simulink model "drone_controller"  (R2026b)
settings: Solver=FixedStepDiscrete  StopTime=0.1  FixedStep=Ts_Rate
model workspace (MAT data in the model file):
  Command_Max = 1
  Kp_Rate = 0.1
  Kp_Tilt = 4
  Quad_X_Mix = [-0.5  0.5  0.5; -0.5  -0.5  -0.5; 0.5  -0.5  0.5; 0.5  0.5  -0.5]
  Quaternion_Norm_Sq_Tol = 0.02
  Rate_Max_radps = 2
  Tilt_Max_rad = 0.436332312999
  Ts_Attitude = 0.01
  Ts_Rate = 0.002
libraries: simulink x6
settings Model: Creator=ASUS  LastModifiedBy=ASUS

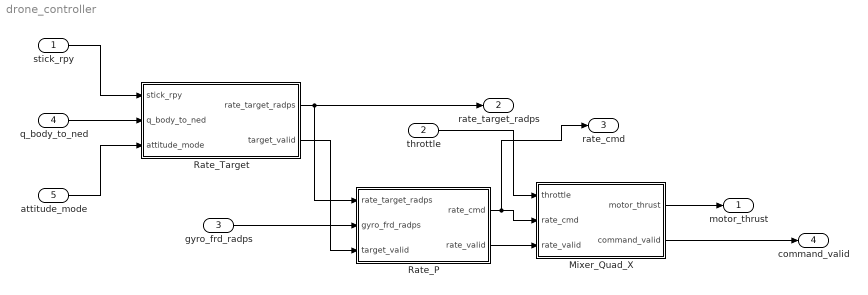
== system drone_controller ==
  stick_rpy : Inport  OutDataTypeStr=double  PortDimensions=3  SampleTime=Ts_Rate  Interpolate=off
  throttle : Inport  Port=2  OutDataTypeStr=double  PortDimensions=1  SampleTime=Ts_Rate  Interpolate=off
  gyro_frd_radps : Inport  Port=3  OutDataTypeStr=double  PortDimensions=3  SampleTime=Ts_Rate  Interpolate=off
  q_body_to_ned : Inport  Port=4  OutDataTypeStr=double  PortDimensions=4  SampleTime=Ts_Rate  Interpolate=off
  attitude_mode : Inport  Port=5  OutDataTypeStr=boolean  PortDimensions=1  SampleTime=Ts_Rate  Interpolate=off
  Mixer_Quad_X : Subsystem
  Rate_P : Subsystem
  Rate_Target : Subsystem
  motor_thrust : Outport
  rate_target_radps : Outport  Port=2
  rate_cmd : Outport  Port=3
  command_valid : Outport  Port=4
  wires:
  stick_rpy/1 -> Rate_Target/1(stick_rpy)
  q_body_to_ned/1 -> Rate_Target/2(q_body_to_ned)
  attitude_mode/1 -> Rate_Target/3(attitude_mode)
  Rate_Target/1(rate_target_radps) -> Rate_P/1(rate_target_radps), rate_target_radps/1
  gyro_frd_radps/1 -> Rate_P/2(gyro_frd_radps)
  Rate_Target/2(target_valid) -> Rate_P/3(target_valid)
  throttle/1 -> Mixer_Quad_X/1(throttle)
  Rate_P/1(rate_cmd) -> Mixer_Quad_X/2(rate_cmd), rate_cmd/1
  Rate_P/2(rate_valid) -> Mixer_Quad_X/3(rate_valid)
  Mixer_Quad_X/1(motor_thrust) -> motor_thrust/1
  Mixer_Quad_X/2(command_valid) -> command_valid/1

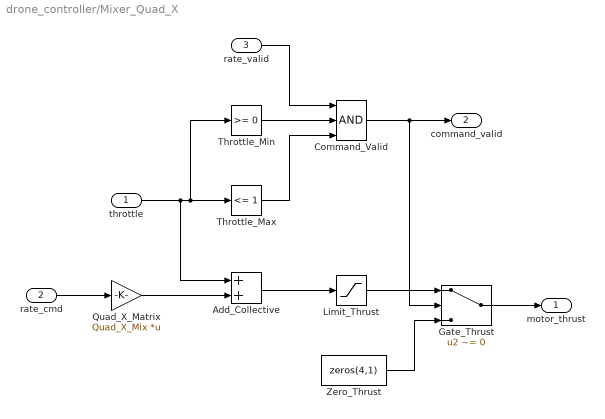
== system drone_controller/Mixer_Quad_X ==
  throttle : Inport
  rate_cmd : Inport  Port=2
  rate_valid : Inport  Port=3
  Add_Collective : Sum
  Command_Valid : Logic  Inputs=3  IconShape=distinctive  AllPortsSameDT=off  OutDataTypeStr=boolean
  Gate_Thrust : Switch  Criteria=u2 ~= 0  SaturateOnIntegerOverflow=off  InputSameDT=off
  Limit_Thrust : Saturate  UpperLimit=1  LowerLimit=0
  Quad_X_Matrix : Gain  Gain=Quad_X_Mix  Multiplication=Matrix(K*u) (u vector)
  Throttle_Max : simulink/Logic and Bit Operations/Compare To Constant  relop=<=  const=1  OutDataTypeStr=boolean
  Throttle_Min : simulink/Logic and Bit Operations/Compare To Constant  relop=>=  const=0  OutDataTypeStr=boolean
  Zero_Thrust : Constant  Value=zeros(4,1)
  motor_thrust : Outport
  command_valid : Outport  Port=2
  wires:
  Gate_Thrust/1 -> motor_thrust/1
  Zero_Thrust/1 -> Gate_Thrust/3
  Command_Valid/1 -> Gate_Thrust/2, command_valid/1
  Limit_Thrust/1 -> Gate_Thrust/1
  Throttle_Max/1 -> Command_Valid/3
  Throttle_Min/1 -> Command_Valid/2
  Add_Collective/1 -> Limit_Thrust/1
  Quad_X_Matrix/1 -> Add_Collective/2
  rate_valid/1 -> Command_Valid/1
  rate_cmd/1 -> Quad_X_Matrix/1
  throttle/1 -> Throttle_Min/1, Throttle_Max/1, Add_Collective/1

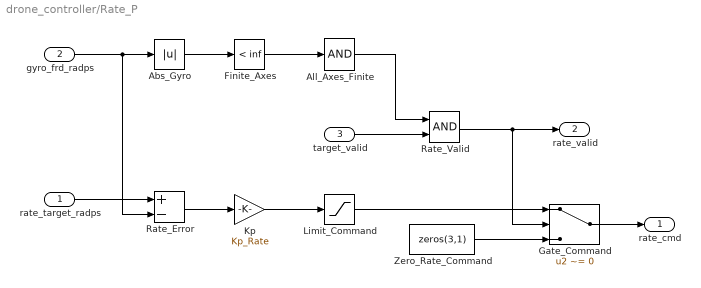
== system drone_controller/Rate_P ==
  rate_target_radps : Inport
  gyro_frd_radps : Inport  Port=2
  target_valid : Inport  Port=3
  Abs_Gyro : Abs  SaturateOnIntegerOverflow=off
  All_Axes_Finite : Logic  Inputs=1  IconShape=distinctive  AllPortsSameDT=off  OutDataTypeStr=boolean
  Finite_Axes : simulink/Logic and Bit Operations/Compare To Constant  relop=<  const=inf  OutDataTypeStr=boolean
  Gate_Command : Switch  Criteria=u2 ~= 0  SaturateOnIntegerOverflow=off  InputSameDT=off
  Kp : Gain  Gain=Kp_Rate
  Limit_Command : Saturate  UpperLimit=Command_Max  LowerLimit=-Command_Max
  Rate_Error : Sum  Inputs=+-
  Rate_Valid : Logic  IconShape=distinctive  AllPortsSameDT=off  OutDataTypeStr=boolean
  Zero_Rate_Command : Constant  Value=zeros(3,1)
  rate_cmd : Outport
  rate_valid : Outport  Port=2
  wires:
  Gate_Command/1 -> rate_cmd/1
  Zero_Rate_Command/1 -> Gate_Command/3
  Limit_Command/1 -> Gate_Command/1
  Rate_Valid/1 -> Gate_Command/2, rate_valid/1
  target_valid/1 -> Rate_Valid/2
  All_Axes_Finite/1 -> Rate_Valid/1
  Finite_Axes/1 -> All_Axes_Finite/1
  Abs_Gyro/1 -> Finite_Axes/1
  Kp/1 -> Limit_Command/1
  Rate_Error/1 -> Kp/1
  gyro_frd_radps/1 -> Rate_Error/2, Abs_Gyro/1
  rate_target_radps/1 -> Rate_Error/1

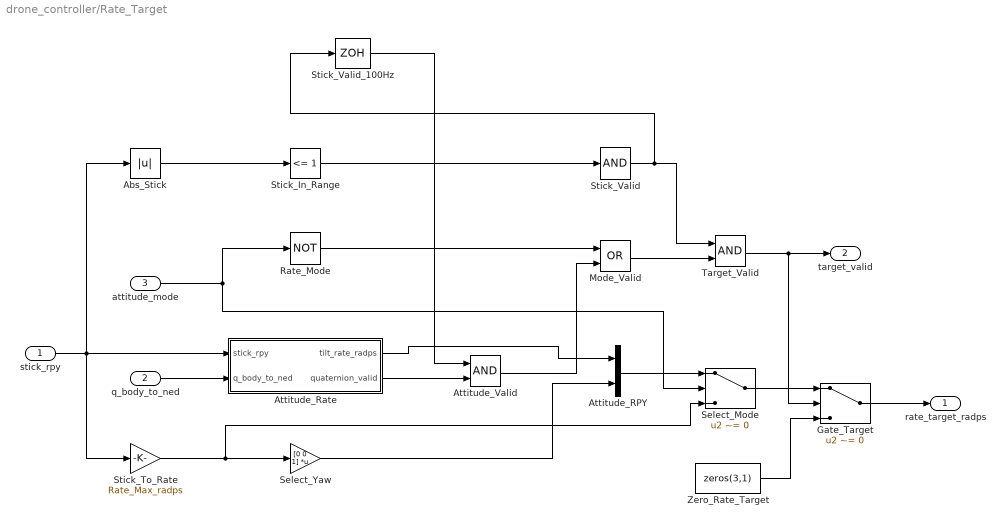
== system drone_controller/Rate_Target ==
  stick_rpy : Inport
  q_body_to_ned : Inport  Port=2
  attitude_mode : Inport  Port=3
  Abs_Stick : Abs  SaturateOnIntegerOverflow=off
  Attitude_RPY : Mux  Inputs=2
  Attitude_Rate : Subsystem
  Attitude_Valid : Logic  AllPortsSameDT=off  OutDataTypeStr=boolean
  Gate_Target : Switch  Criteria=u2 ~= 0  SaturateOnIntegerOverflow=off  InputSameDT=off
  Mode_Valid : Logic  Operator=OR  IconShape=distinctive  AllPortsSameDT=off  OutDataTypeStr=boolean
  Rate_Mode : Logic  Operator=NOT  Inputs=1  IconShape=distinctive  AllPortsSameDT=off  OutDataTypeStr=boolean
  Select_Mode : Switch  Criteria=u2 ~= 0  SaturateOnIntegerOverflow=off  InputSameDT=off
  Select_Yaw : Gain  Gain=[0 0 1]  Multiplication=Matrix(K*u) (u vector)
  Stick_In_Range : simulink/Logic and Bit Operations/Compare To Constant  relop=<=  const=1  OutDataTypeStr=boolean
  Stick_To_Rate : Gain  Gain=Rate_Max_radps
  Stick_Valid : Logic  Inputs=1  IconShape=distinctive  AllPortsSameDT=off  OutDataTypeStr=boolean
  Stick_Valid_100Hz : ZeroOrderHold  SampleTime=Ts_Attitude
  Target_Valid : Logic  IconShape=distinctive  AllPortsSameDT=off  OutDataTypeStr=boolean
  Zero_Rate_Target : Constant  Value=zeros(3,1)
  rate_target_radps : Outport
  target_valid : Outport  Port=2
  wires:
  Gate_Target/1 -> rate_target_radps/1
  Zero_Rate_Target/1 -> Gate_Target/3
  Target_Valid/1 -> Gate_Target/2, target_valid/1
  Select_Mode/1 -> Gate_Target/1
  Mode_Valid/1 -> Target_Valid/2
  Rate_Mode/1 -> Mode_Valid/1
  Stick_In_Range/1 -> Stick_Valid/1
  Abs_Stick/1 -> Stick_In_Range/1
  Attitude_RPY/1 -> Select_Mode/1
  Select_Yaw/1 -> Attitude_RPY/2
  Stick_To_Rate/1 -> Select_Yaw/1, Select_Mode/3
  attitude_mode/1 -> Select_Mode/2, Rate_Mode/1
  q_body_to_ned/1 -> Attitude_Rate/2(q_body_to_ned)
  stick_rpy/1 -> Attitude_Rate/1(stick_rpy), Stick_To_Rate/1, Abs_Stick/1
  Attitude_Valid/1 -> Mode_Valid/2
  Stick_Valid_100Hz/1 -> Attitude_Valid/1
  Attitude_Rate/1(tilt_rate_radps) -> Attitude_RPY/1
  Stick_Valid/1 -> Stick_Valid_100Hz/1, Target_Valid/1
  Attitude_Rate/2(quaternion_valid) -> Attitude_Valid/2

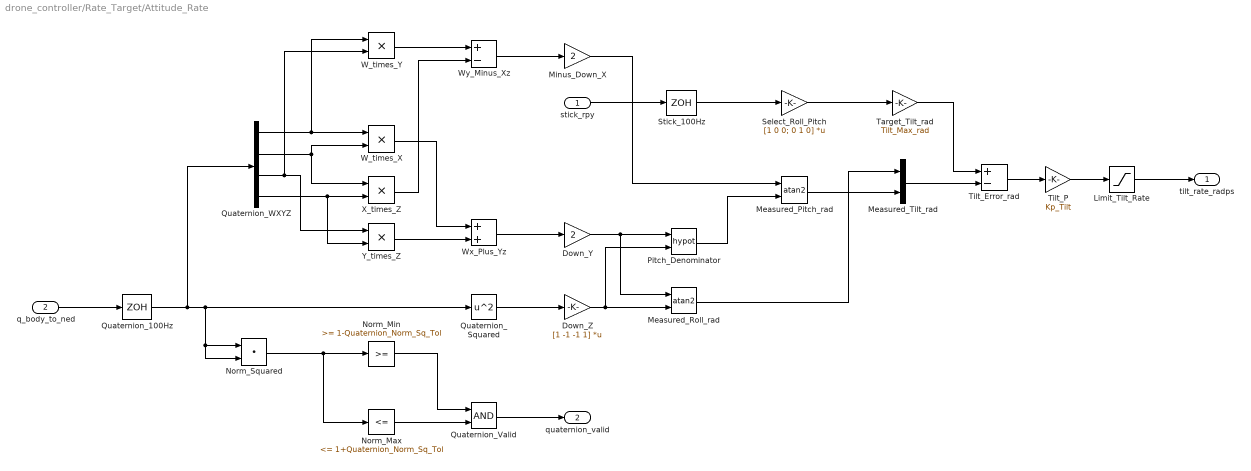
== system drone_controller/Rate_Target/Attitude_Rate ==
  stick_rpy : Inport
  q_body_to_ned : Inport  Port=2
  Down_Y : Gain  Gain=2
  Down_Z : Gain  Gain=[1 -1 -1 1]  Multiplication=Matrix(K*u) (u vector)
  Limit_Tilt_Rate : Saturate  UpperLimit=Rate_Max_radps  LowerLimit=-Rate_Max_radps
  Measured_Pitch_rad : Trigonometry  Operator=atan2
  Measured_Roll_rad : Trigonometry  Operator=atan2
  Measured_Tilt_rad : Mux  Inputs=2
  Minus_Down_X : Gain  Gain=2
  Norm_Max : simulink/Logic and Bit Operations/Compare To Constant  relop=<=  const=1+Quaternion_Norm_Sq_Tol  OutDataTypeStr=boolean
  Norm_Min : simulink/Logic and Bit Operations/Compare To Constant  relop=>=  const=1-Quaternion_Norm_Sq_Tol  OutDataTypeStr=boolean
  Norm_Squared : DotProduct  OutDataTypeStr=Inherit: Inherit via internal rule
  Pitch_Denominator : Math  Operator=hypot
  Quaternion_100Hz : ZeroOrderHold  SampleTime=Ts_Attitude
  Quaternion_Squared : Math  Operator=square
  Quaternion_Valid : Logic  IconShape=distinctive  AllPortsSameDT=off  OutDataTypeStr=boolean
  Quaternion_WXYZ : Demux
  Select_Roll_Pitch : Gain  Gain=[1 0 0; 0 1 0]  Multiplication=Matrix(K*u) (u vector)
  Stick_100Hz : ZeroOrderHold  SampleTime=Ts_Attitude
  Target_Tilt_rad : Gain  Gain=Tilt_Max_rad
  Tilt_Error_rad : Sum  Inputs=+-
  Tilt_P : Gain  Gain=Kp_Tilt
  W_times_X : Product  Inputs=**
  W_times_Y : Product  Inputs=**
  Wx_Plus_Yz : Sum
  Wy_Minus_Xz : Sum  Inputs=+-
  X_times_Z : Product  Inputs=**
  Y_times_Z : Product  Inputs=**
  tilt_rate_radps : Outport
  quaternion_valid : Outport  Port=2
  wires:
  Limit_Tilt_Rate/1 -> tilt_rate_radps/1
  Tilt_P/1 -> Limit_Tilt_Rate/1
  Tilt_Error_rad/1 -> Tilt_P/1
  Measured_Tilt_rad/1 -> Tilt_Error_rad/2
  Target_Tilt_rad/1 -> Tilt_Error_rad/1
  Measured_Pitch_rad/1 -> Measured_Tilt_rad/2
  Measured_Roll_rad/1 -> Measured_Tilt_rad/1
  Pitch_Denominator/1 -> Measured_Pitch_rad/2
  Minus_Down_X/1 -> Measured_Pitch_rad/1
  Down_Z/1 -> Measured_Roll_rad/2, Pitch_Denominator/2
  Down_Y/1 -> Measured_Roll_rad/1, Pitch_Denominator/1
  Quaternion_Squared/1 -> Down_Z/1
  Wy_Minus_Xz/1 -> Minus_Down_X/1
  Wx_Plus_Yz/1 -> Down_Y/1
  X_times_Z/1 -> Wy_Minus_Xz/2
  W_times_Y/1 -> Wy_Minus_Xz/1
  Y_times_Z/1 -> Wx_Plus_Yz/2
  W_times_X/1 -> Wx_Plus_Yz/1
  Quaternion_WXYZ/4 -> Y_times_Z/2, X_times_Z/2
  Quaternion_WXYZ/3 -> Y_times_Z/1, W_times_Y/2
  Quaternion_WXYZ/2 -> W_times_X/2, X_times_Z/1
  Quaternion_WXYZ/1 -> W_times_X/1, W_times_Y/1
  Quaternion_Valid/1 -> quaternion_valid/1
  Norm_Max/1 -> Quaternion_Valid/2
  Norm_Min/1 -> Quaternion_Valid/1
  Norm_Squared/1 -> Norm_Min/1, Norm_Max/1
  Quaternion_100Hz/1 -> Norm_Squared/2, Norm_Squared/1, Quaternion_Squared/1, Quaternion_WXYZ/1
  Select_Roll_Pitch/1 -> Target_Tilt_rad/1
  Stick_100Hz/1 -> Select_Roll_Pitch/1
  q_body_to_ned/1 -> Quaternion_100Hz/1
  stick_rpy/1 -> Stick_100Hz/1
